simulink model "foc_simulink"  (R2022b)
settings: Solver=FixedStepDiscrete  StartTime=0.0  StopTime=0.5  RelTol=1e-3
InitFcn:
  | SPEED_PI_P=0.003
  | SPEED_PI_I=5
  | SPEED_PI_UP_LIMIT = 5.0
  | SPEED_PI_LOW_LIMIT = -5.0
  | SPEED_PI_KB = 0.015
  | D_PI_P = 1.4
  | D_PI_I = 600
  | D_PI_UP_LIMIT = 24.0
  | D_PI_LOW_LIMIT = -24.0
  | D_PI_KB = 15
  | Q_PI_P = 1.4
  | Q_PI_I = 600
  | Q_PI_UP_LIMIT = 24.0
  | Q_PI_LOW_LIMIT = -24.0
  | Q_PI_KB = 15
values from neighbouring files (symbols this model uses):
  L = 0.00046    [electric_current_loop.m]    (also in electric_kp_ki.m; pll.m = 10000; sl_ekf.m = c.L_LINE; sl_flux.m = L_avg - 0.5 * L_diff + L_diff * iq_obs * iq_obs / i2_obs)
libraries: slpidlib x8, spsPermanentMagnetSynchronousMachineLib x3, simulink x2, spsDCVoltageSourceLib x1, spsGroundLib x1, spsThreePhaseVIMeasurementLib x1, spsUniversalBridgeLib x1, sps_lib x1
(part 2 of 2)

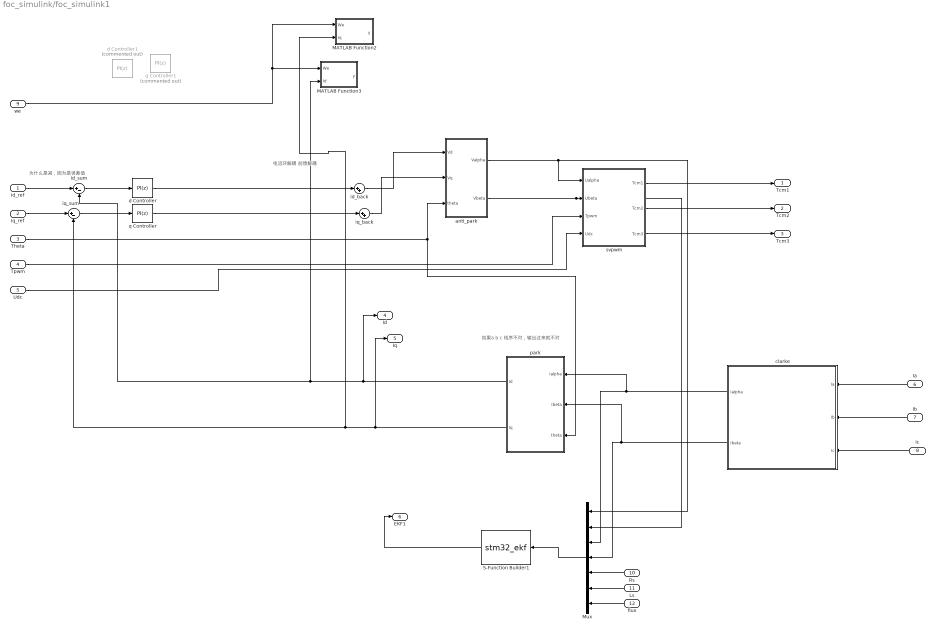
== system foc_simulink/foc_simulink1 ==
  note: 如果a b c 线序不对，输出过来就不对
  note: 为什么是减，因为是误差值
  note: 电流环解耦
      | 前馈解耦
  Id_ref : Inport
  Iq_ref : Inport  Port=2
  Theta : Inport  Port=3
  Tpwm : Inport  Port=4
  Udc : Inport  Port=5
  Ia : Inport  Port=6
  Ib : Inport  Port=7
  Ic : Inport  Port=8
  we : Inport  Port=9
  Rs : Inport  Port=10
  Ls : Inport  Port=11
  flux : Inport  Port=12
  MATLAB Function2 : MATLAB Function  TreatAsAtomicUnit=on
  MATLAB Function3 : MATLAB Function  TreatAsAtomicUnit=on
  Mux : Mux  Inputs=7
  S-Function Builder1 : S-Function  InitFcn=try, set_param(gcb,'FunctionName','stm32_ekf'), end  FunctionName=stm32_ekf  SFunctionModules=stm32_ekf_wrapper  SFunctionDeploymentMode=off  EnableBusSupport=off  mask(S-Function Builder){}
      mask help: Simulink:masks:SFunctionBuilder_MD
      mask init: same as foc_simulink/foc_simulink/EKF
      settings: CopyFcn=set_param(gcbh,'LinkStatus','none')  PreSaveFcn=try, set_param(gcb,'FunctionName','stm32_ekf'), end  OpenFcn=sfunctionwizard(gcbh)
      mask Display: plot(val(:,1),val(:,2)),disp(sys), port_label('input',1,'u'), port_label('output',1,'y')
  anti_park : Subsystem
  clarke : Subsystem
  d Controller : slpidlib/PID Controller  Controller=PI  Form=Parallel  TimeDomain=Discrete-time  UseExternalTs=off  SampleTime=-1  IntegratorMethod=Forward Euler  FilterMethod=Forward Euler  ControllerParametersSource=internal  P=D_PI_P  I=D_PI_I  UseKiTs=off  D=0.09  N=100  UseFilter=on  TunerSelectOption=Transfer Function Based (PID Tuner App)  InitialConditionSource=internal  InitialConditionForIntegrator=0  InitialConditionForFilter=0  DifferentiatorICPrevScaledInput=0  ExternalReset=none  TrackingMode=off  Kt=1  LimitOutput=on  SatLimitsSource=internal  UpperSaturationLimit=D_PI_UP_LIMIT  LowerSaturationLimit=D_PI_LOW_LIMIT  LinearizeAsGain=off  AntiWindupMode=back-calculation  Kb=D_PI_KB  LimitIntegrator=off  UpperIntegratorSaturationLimit=inf  LowerIntegratorSaturationLimit=-inf  PGainOutDataTypeStr=single  PProdOutDataTypeStr=single  POutMin=[]  POutMax=[]  IGainOutDataTypeStr=single  IProdOutDataTypeStr=single  IOutMin=[]  IOutMax=[]  DOutMin=[]  DOutMax=[]  NOutMin=[]  NOutMax=[]  SumOutDataTypeStr=single  SumOutMin=[]  SumOutMax=[]  SaturationOutDataTypeStr=single  SaturationOutMin=[]  SaturationOutMax=[]  PParamDataTypeStr=single  PParamMin=[]  PParamMax=[]  IParamDataTypeStr=single  IParamMin=[]  IParamMax=[]  DParamMin=[]  DParamMax=[]  NParamMin=[]  NParamMax=[]  KbParamDataTypeStr=single  KbParamMin=[]  KbParamMax=[]  KtParamMin=[]  KtParamMax=[]  KbOutDataTypeStr=single  KbOutMin=[]  KbOutMax=[]  KtOutMin=[]  KtOutMax=[]  IntegratorOutDataTypeStr=single  IntegratorOutMin=[]  IntegratorOutMax=[]  FilterOutMin=[]  FilterOutMax=[]  SumI1OutDataTypeStr=single  SumI1OutMin=[]  SumI1OutMax=[]  SumI2OutDataTypeStr=single  SumI2OutMin=[]  SumI2OutMax=[]  SumI3OutMin=[]  SumI3OutMax=[]  SumI4OutMin=[]  SumI4OutMax=[]  SumDOutMin=[]  SumDOutMax=[]  SumAccumDataTypeStr=single  SumI1AccumDataTypeStr=single  SumI2AccumDataTypeStr=single  DifferentiatorOutMin=[]  DifferentiatorOutMax=[]  FilterDiffOutCoefMin=[]  FilterDiffOutCoefMax=[]  ReciprocalOutMin=[]  ReciprocalOutMax=[]  SumDenOutMin=[]  SumDenOutMax=[]  SumNumOutMin=[]  SumNumOutMax=[]  DivideOutMin=[]  DivideOutMax=[]  UdiffTsProdOutMin=[]  UdiffTsProdOutMax=[]  NTsProdOutMin=[]  NTsProdOutMax=[]  UintegralTsProdOutMin=[]  UintegralTsProdOutMax=[]  UngainTsProdOutMin=[]  UngainTsProdOutMax=[]  ClampingZeroOutDataTypeStr=Inherit: Inherit via back propagation  ClampingZeroOutMin=[]  ClampingZeroOutMax=[]  FilterDenConstantOutDataTypeStr=Inherit: Inherit via back propagation  FilterDenConstantOutMin=[]  FilterDenConstantOutMax=[]  PCopyOutDataTypeStr=Inherit: Inherit via back propagation  PCopyOutMin=[]  PCopyOutMax=[]  NCopyOutDataTypeStr=Inherit: Inherit via back propagation  NCopyOutMin=[]  NCopyOutMax=[]  IntegratorContinuousStateAttributes=''  IntegratorStateIdentifier=di  IntegratorStateMustResolveToSignalObject=off  IntegratorRTWStateStorageClass=Auto  FilterContinuousStateAttributes=''  FilterStateMustResolveToSignalObject=off  FilterRTWStateStorageClass=Auto  ParallelPVariant=InternalParameters  IdealPVariant=Disabled  IVariant=InternalParameters  DVariant=Disabled  IntegratorVariant=Discrete  SatVariant=Enabled  AWVariant=BackCalculation  PCopyVariant=Disabled  TRVariant=Disabled  FdbkBlocksVariant=Forward  IdealPFdbkVariant=Disabled  SatFdbkVariant=Disabled  DerivativeFilterVariant=Disabled  NVariant=Disabled  NCopyVariant=Disabled_SignalSpec  FilterICVariant=Disabled  IntegratorICVariant=InternalICs  ExternalResetVariant=Disabled  TRSumVariant=Passthrough  SumFdbkVariant=Disabled  SumVariant=Sum_PI  TsampFilterVariant=InternalTs  TsampNgainVariant=Passthrough  TsampIntegralVariant=Passthrough  ExternalSaturationOutDataTypeStr=Inherit: Same as second input
  d Controller1 : slpidlib/PID Controller  Commented=on  Controller=PI  Form=Parallel  TimeDomain=Discrete-time  UseExternalTs=off  SampleTime=-1  IntegratorMethod=Forward Euler  FilterMethod=Forward Euler  ControllerParametersSource=internal  P=D_PI_P  I=D_PI_I  UseKiTs=off  D=0.09  N=100  UseFilter=on  TunerSelectOption=Transfer Function Based (PID Tuner App)  InitialConditionSource=internal  InitialConditionForIntegrator=0  InitialConditionForFilter=0  DifferentiatorICPrevScaledInput=0  ExternalReset=none  TrackingMode=off  Kt=1  LimitOutput=on  SatLimitsSource=internal  UpperSaturationLimit=D_PI_UP_LIMIT  LowerSaturationLimit=D_PI_LOW_LIMIT  LinearizeAsGain=off  AntiWindupMode=back-calculation  Kb=D_PI_KB  LimitIntegrator=off  UpperIntegratorSaturationLimit=inf  LowerIntegratorSaturationLimit=-inf  PGainOutDataTypeStr=single  PProdOutDataTypeStr=single  POutMin=[]  POutMax=[]  IGainOutDataTypeStr=single  IProdOutDataTypeStr=single  IOutMin=[]  IOutMax=[]  DOutMin=[]  DOutMax=[]  NOutMin=[]  NOutMax=[]  SumOutDataTypeStr=single  SumOutMin=[]  SumOutMax=[]  SaturationOutDataTypeStr=single  SaturationOutMin=[]  SaturationOutMax=[]  PParamDataTypeStr=single  PParamMin=[]  PParamMax=[]  IParamDataTypeStr=single  IParamMin=[]  IParamMax=[]  DParamMin=[]  DParamMax=[]  NParamMin=[]  NParamMax=[]  KbParamDataTypeStr=single  KbParamMin=[]  KbParamMax=[]  KtParamMin=[]  KtParamMax=[]  KbOutDataTypeStr=single  KbOutMin=[]  KbOutMax=[]  KtOutMin=[]  KtOutMax=[]  IntegratorOutDataTypeStr=single  IntegratorOutMin=[]  IntegratorOutMax=[]  FilterOutMin=[]  FilterOutMax=[]  SumI1OutDataTypeStr=single  SumI1OutMin=[]  SumI1OutMax=[]  SumI2OutDataTypeStr=single  SumI2OutMin=[]  SumI2OutMax=[]  SumI3OutMin=[]  SumI3OutMax=[]  SumI4OutMin=[]  SumI4OutMax=[]  SumDOutMin=[]  SumDOutMax=[]  SumAccumDataTypeStr=single  SumI1AccumDataTypeStr=single  SumI2AccumDataTypeStr=single  DifferentiatorOutMin=[]  DifferentiatorOutMax=[]  FilterDiffOutCoefMin=[]  FilterDiffOutCoefMax=[]  ReciprocalOutMin=[]  ReciprocalOutMax=[]  SumDenOutMin=[]  SumDenOutMax=[]  SumNumOutMin=[]  SumNumOutMax=[]  DivideOutMin=[]  DivideOutMax=[]  UdiffTsProdOutMin=[]  UdiffTsProdOutMax=[]  NTsProdOutMin=[]  NTsProdOutMax=[]  UintegralTsProdOutMin=[]  UintegralTsProdOutMax=[]  UngainTsProdOutMin=[]  UngainTsProdOutMax=[]  ClampingZeroOutDataTypeStr=Inherit: Inherit via back propagation  ClampingZeroOutMin=[]  ClampingZeroOutMax=[]  FilterDenConstantOutDataTypeStr=Inherit: Inherit via back propagation  FilterDenConstantOutMin=[]  FilterDenConstantOutMax=[]  PCopyOutDataTypeStr=Inherit: Inherit via back propagation  PCopyOutMin=[]  PCopyOutMax=[]  NCopyOutDataTypeStr=Inherit: Inherit via back propagation  NCopyOutMin=[]  NCopyOutMax=[]  IntegratorContinuousStateAttributes=''  IntegratorStateIdentifier=di  IntegratorStateMustResolveToSignalObject=off  IntegratorRTWStateStorageClass=Auto  FilterContinuousStateAttributes=''  FilterStateMustResolveToSignalObject=off  FilterRTWStateStorageClass=Auto  ParallelPVariant=InternalParameters  IdealPVariant=Disabled  IVariant=InternalParameters  DVariant=Disabled  IntegratorVariant=Discrete  SatVariant=Enabled  AWVariant=BackCalculation  PCopyVariant=Disabled  TRVariant=Disabled  FdbkBlocksVariant=Forward  IdealPFdbkVariant=Disabled  SatFdbkVariant=Disabled  DerivativeFilterVariant=Disabled  NVariant=Disabled  NCopyVariant=Disabled_SignalSpec  FilterICVariant=Disabled  IntegratorICVariant=InternalICs  ExternalResetVariant=Disabled  TRSumVariant=Passthrough  SumFdbkVariant=Disabled  SumVariant=Sum_PI  TsampFilterVariant=InternalTs  TsampNgainVariant=Passthrough  TsampIntegralVariant=Passthrough  ExternalSaturationOutDataTypeStr=Inherit: Same as second input
  id_back : Sum  Inputs=|++
  id_sum : Sum  Inputs=|+-
  iq_back : Sum  Inputs=|++
  iq_sum : Sum  Inputs=|+-
  park : Subsystem
  q Controller : slpidlib/PID Controller  Controller=PI  Form=Parallel  TimeDomain=Discrete-time  UseExternalTs=off  SampleTime=-1  IntegratorMethod=Forward Euler  FilterMethod=Forward Euler  ControllerParametersSource=internal  P=Q_PI_P  I=Q_PI_I  UseKiTs=off  D=0.09  N=100  UseFilter=on  TunerSelectOption=Transfer Function Based (PID Tuner App)  InitialConditionSource=internal  InitialConditionForIntegrator=0  InitialConditionForFilter=0  DifferentiatorICPrevScaledInput=0  ExternalReset=none  TrackingMode=off  Kt=1  LimitOutput=on  SatLimitsSource=internal  UpperSaturationLimit=Q_PI_UP_LIMIT  LowerSaturationLimit=Q_PI_LOW_LIMIT  LinearizeAsGain=off  AntiWindupMode=back-calculation  Kb=Q_PI_KB  LimitIntegrator=off  UpperIntegratorSaturationLimit=inf  LowerIntegratorSaturationLimit=-inf  PGainOutDataTypeStr=single  PProdOutDataTypeStr=single  POutMin=[]  POutMax=[]  IGainOutDataTypeStr=single  IProdOutDataTypeStr=single  IOutMin=[]  IOutMax=[]  DOutMin=[]  DOutMax=[]  NOutMin=[]  NOutMax=[]  SumOutDataTypeStr=single  SumOutMin=[]  SumOutMax=[]  SaturationOutDataTypeStr=single  SaturationOutMin=[]  SaturationOutMax=[]  PParamDataTypeStr=single  PParamMin=[]  PParamMax=[]  IParamDataTypeStr=single  IParamMin=[]  IParamMax=[]  DParamMin=[]  DParamMax=[]  NParamMin=[]  NParamMax=[]  KbParamDataTypeStr=single  KbParamMin=[]  KbParamMax=[]  KtParamMin=[]  KtParamMax=[]  KbOutDataTypeStr=single  KbOutMin=[]  KbOutMax=[]  KtOutMin=[]  KtOutMax=[]  IntegratorOutDataTypeStr=single  IntegratorOutMin=[]  IntegratorOutMax=[]  FilterOutMin=[]  FilterOutMax=[]  SumI1OutDataTypeStr=single  SumI1OutMin=[]  SumI1OutMax=[]  SumI2OutDataTypeStr=single  SumI2OutMin=[]  SumI2OutMax=[]  SumI3OutMin=[]  SumI3OutMax=[]  SumI4OutMin=[]  SumI4OutMax=[]  SumDOutMin=[]  SumDOutMax=[]  SumAccumDataTypeStr=single  SumI1AccumDataTypeStr=single  SumI2AccumDataTypeStr=single  DifferentiatorOutMin=[]  DifferentiatorOutMax=[]  FilterDiffOutCoefMin=[]  FilterDiffOutCoefMax=[]  ReciprocalOutMin=[]  ReciprocalOutMax=[]  SumDenOutMin=[]  SumDenOutMax=[]  SumNumOutMin=[]  SumNumOutMax=[]  DivideOutMin=[]  DivideOutMax=[]  UdiffTsProdOutMin=[]  UdiffTsProdOutMax=[]  NTsProdOutMin=[]  NTsProdOutMax=[]  UintegralTsProdOutMin=[]  UintegralTsProdOutMax=[]  UngainTsProdOutMin=[]  UngainTsProdOutMax=[]  ClampingZeroOutDataTypeStr=Inherit: Inherit via back propagation  ClampingZeroOutMin=[]  ClampingZeroOutMax=[]  FilterDenConstantOutDataTypeStr=Inherit: Inherit via back propagation  FilterDenConstantOutMin=[]  FilterDenConstantOutMax=[]  PCopyOutDataTypeStr=Inherit: Inherit via back propagation  PCopyOutMin=[]  PCopyOutMax=[]  NCopyOutDataTypeStr=Inherit: Inherit via back propagation  NCopyOutMin=[]  NCopyOutMax=[]  IntegratorContinuousStateAttributes=''  IntegratorStateIdentifier=qi  IntegratorStateMustResolveToSignalObject=off  IntegratorRTWStateStorageClass=Auto  FilterContinuousStateAttributes=''  FilterStateMustResolveToSignalObject=off  FilterRTWStateStorageClass=Auto  ParallelPVariant=InternalParameters  IdealPVariant=Disabled  IVariant=InternalParameters  DVariant=Disabled  IntegratorVariant=Discrete  SatVariant=Enabled  AWVariant=BackCalculation  PCopyVariant=Disabled  TRVariant=Disabled  FdbkBlocksVariant=Forward  IdealPFdbkVariant=Disabled  SatFdbkVariant=Disabled  DerivativeFilterVariant=Disabled  NVariant=Disabled  NCopyVariant=Disabled_SignalSpec  FilterICVariant=Disabled  IntegratorICVariant=InternalICs  ExternalResetVariant=Disabled  TRSumVariant=Passthrough  SumFdbkVariant=Disabled  SumVariant=Sum_PI  TsampFilterVariant=InternalTs  TsampNgainVariant=Passthrough  TsampIntegralVariant=Passthrough  ExternalSaturationOutDataTypeStr=Inherit: Same as second input
  q Controller1 : slpidlib/PID Controller  Commented=on  Controller=PI  Form=Parallel  TimeDomain=Discrete-time  UseExternalTs=off  SampleTime=-1  IntegratorMethod=Forward Euler  FilterMethod=Forward Euler  ControllerParametersSource=internal  P=Q_PI_P  I=Q_PI_I  UseKiTs=off  D=0.09  N=100  UseFilter=on  TunerSelectOption=Transfer Function Based (PID Tuner App)  InitialConditionSource=internal  InitialConditionForIntegrator=0  InitialConditionForFilter=0  DifferentiatorICPrevScaledInput=0  ExternalReset=none  TrackingMode=off  Kt=1  LimitOutput=on  SatLimitsSource=internal  UpperSaturationLimit=Q_PI_UP_LIMIT  LowerSaturationLimit=Q_PI_LOW_LIMIT  LinearizeAsGain=off  AntiWindupMode=back-calculation  Kb=Q_PI_KB  LimitIntegrator=off  UpperIntegratorSaturationLimit=inf  LowerIntegratorSaturationLimit=-inf  PGainOutDataTypeStr=single  PProdOutDataTypeStr=single  POutMin=[]  POutMax=[]  IGainOutDataTypeStr=single  IProdOutDataTypeStr=single  IOutMin=[]  IOutMax=[]  DOutMin=[]  DOutMax=[]  NOutMin=[]  NOutMax=[]  SumOutDataTypeStr=single  SumOutMin=[]  SumOutMax=[]  SaturationOutDataTypeStr=single  SaturationOutMin=[]  SaturationOutMax=[]  PParamDataTypeStr=single  PParamMin=[]  PParamMax=[]  IParamDataTypeStr=single  IParamMin=[]  IParamMax=[]  DParamMin=[]  DParamMax=[]  NParamMin=[]  NParamMax=[]  KbParamDataTypeStr=single  KbParamMin=[]  KbParamMax=[]  KtParamMin=[]  KtParamMax=[]  KbOutDataTypeStr=single  KbOutMin=[]  KbOutMax=[]  KtOutMin=[]  KtOutMax=[]  IntegratorOutDataTypeStr=single  IntegratorOutMin=[]  IntegratorOutMax=[]  FilterOutMin=[]  FilterOutMax=[]  SumI1OutDataTypeStr=single  SumI1OutMin=[]  SumI1OutMax=[]  SumI2OutDataTypeStr=single  SumI2OutMin=[]  SumI2OutMax=[]  SumI3OutMin=[]  SumI3OutMax=[]  SumI4OutMin=[]  SumI4OutMax=[]  SumDOutMin=[]  SumDOutMax=[]  SumAccumDataTypeStr=single  SumI1AccumDataTypeStr=single  SumI2AccumDataTypeStr=single  DifferentiatorOutMin=[]  DifferentiatorOutMax=[]  FilterDiffOutCoefMin=[]  FilterDiffOutCoefMax=[]  ReciprocalOutMin=[]  ReciprocalOutMax=[]  SumDenOutMin=[]  SumDenOutMax=[]  SumNumOutMin=[]  SumNumOutMax=[]  DivideOutMin=[]  DivideOutMax=[]  UdiffTsProdOutMin=[]  UdiffTsProdOutMax=[]  NTsProdOutMin=[]  NTsProdOutMax=[]  UintegralTsProdOutMin=[]  UintegralTsProdOutMax=[]  UngainTsProdOutMin=[]  UngainTsProdOutMax=[]  ClampingZeroOutDataTypeStr=Inherit: Inherit via back propagation  ClampingZeroOutMin=[]  ClampingZeroOutMax=[]  FilterDenConstantOutDataTypeStr=Inherit: Inherit via back propagation  FilterDenConstantOutMin=[]  FilterDenConstantOutMax=[]  PCopyOutDataTypeStr=Inherit: Inherit via back propagation  PCopyOutMin=[]  PCopyOutMax=[]  NCopyOutDataTypeStr=Inherit: Inherit via back propagation  NCopyOutMin=[]  NCopyOutMax=[]  IntegratorContinuousStateAttributes=''  IntegratorStateIdentifier=qi  IntegratorStateMustResolveToSignalObject=off  IntegratorRTWStateStorageClass=Auto  FilterContinuousStateAttributes=''  FilterStateMustResolveToSignalObject=off  FilterRTWStateStorageClass=Auto  ParallelPVariant=InternalParameters  IdealPVariant=Disabled  IVariant=InternalParameters  DVariant=Disabled  IntegratorVariant=Discrete  SatVariant=Enabled  AWVariant=BackCalculation  PCopyVariant=Disabled  TRVariant=Disabled  FdbkBlocksVariant=Forward  IdealPFdbkVariant=Disabled  SatFdbkVariant=Disabled  DerivativeFilterVariant=Disabled  NVariant=Disabled  NCopyVariant=Disabled_SignalSpec  FilterICVariant=Disabled  IntegratorICVariant=InternalICs  ExternalResetVariant=Disabled  TRSumVariant=Passthrough  SumFdbkVariant=Disabled  SumVariant=Sum_PI  TsampFilterVariant=InternalTs  TsampNgainVariant=Passthrough  TsampIntegralVariant=Passthrough  ExternalSaturationOutDataTypeStr=Inherit: Same as second input
  svpwm : Subsystem
  Tcm1 : Outport
  Tcm2 : Outport  Port=2
  Tcm3 : Outport  Port=3
  Id : Outport  Port=4
  Iq : Outport  Port=5
  EKF1 : Outport  Port=6  VectorParamsAs1DForOutWhenUnconnected=off
  wires:
  flux/1 -> Mux/7
  S-Function Builder1/1 -> EKF1/1
  anti_park/2(Vbeta) -> svpwm/2(Ubeta), Mux/2
  clarke/2(Ibeta) -> park/2(Ibeta), Mux/4
  clarke/1(Ialpha) -> Mux/3, park/1(Ialpha)
  Mux/1 -> S-Function Builder1/1
  anti_park/1(Valpha) -> svpwm/1(Ualpha), Mux/1
  Rs/1 -> Mux/5
  Ls/1 -> Mux/6
  iq_back/1 -> anti_park/2(Vq)
  id_back/1 -> anti_park/1(Vd)
  d Controller/1 -> id_back/1
  id_sum/1 -> d Controller/1
  Id_ref/1 -> id_sum/1
  q Controller/1 -> iq_back/1
  we/1 -> MATLAB Function2/1(We), MATLAB Function3/1(We)
  iq_sum/1 -> q Controller/1
  Iq_ref/1 -> iq_sum/1
  park/2(Iq) -> iq_sum/2, MATLAB Function2/2(Iq), Iq/1
  park/1(Id) -> id_sum/2, MATLAB Function3/2(Id), Id/1
  Ic/1 -> clarke/3(Ic)
  Ib/1 -> clarke/2(Ib)
  Ia/1 -> clarke/1(Ia)
  svpwm/2(Tcm2) -> Tcm2/1
  svpwm/1(Tcm1) -> Tcm1/1
  svpwm/3(Tcm3) -> Tcm3/1
  Tpwm/1 -> svpwm/3(Tpwm)
  Udc/1 -> svpwm/4(Udc)
  Theta/1 -> park/3(theta), anti_park/3(theta)

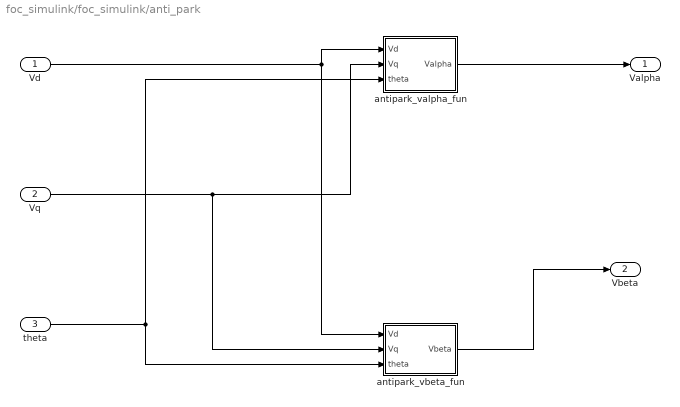
== system foc_simulink/foc_simulink/anti_park ==
  Vd : Inport
  Vq : Inport  Port=2
  theta : Inport  Port=3
  antipark_valpha_fun : MATLAB Function  TreatAsAtomicUnit=on
  antipark_vbeta_fun : MATLAB Function  TreatAsAtomicUnit=on
  Valpha : Outport
  Vbeta : Outport  Port=2
  wires:
  antipark_valpha_fun/1(Valpha) -> Valpha/1
  antipark_vbeta_fun/1(Vbeta) -> Vbeta/1
  Vd/1 -> antipark_valpha_fun/1(Vd), antipark_vbeta_fun/1(Vd)
  Vq/1 -> antipark_valpha_fun/2(Vq), antipark_vbeta_fun/2(Vq)
  theta/1 -> antipark_valpha_fun/3(theta), antipark_vbeta_fun/3(theta)

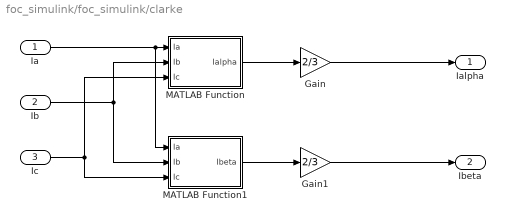
== system foc_simulink/foc_simulink/clarke ==
  Ia : Inport
  Ib : Inport  Port=2
  Ic : Inport  Port=3
  Gain : Gain  Gain=2/3  OutDataTypeStr=single
  Gain1 : Gain  Gain=2/3  OutDataTypeStr=single
  MATLAB Function : MATLAB Function  TreatAsAtomicUnit=on
  MATLAB Function1 : MATLAB Function  TreatAsAtomicUnit=on
  Ialpha : Outport
  Ibeta : Outport  Port=2
  wires:
  Ia/1 -> MATLAB Function1/1(Ia), MATLAB Function/1(Ia)
  MATLAB Function/1(Ialpha) -> Gain/1
  Gain1/1 -> Ibeta/1
  Ib/1 -> MATLAB Function1/2(Ib), MATLAB Function/2(Ib)
  Ic/1 -> MATLAB Function/3(Ic), MATLAB Function1/3(Ic)
  MATLAB Function1/1(Ibeta) -> Gain1/1
  Gain/1 -> Ialpha/1

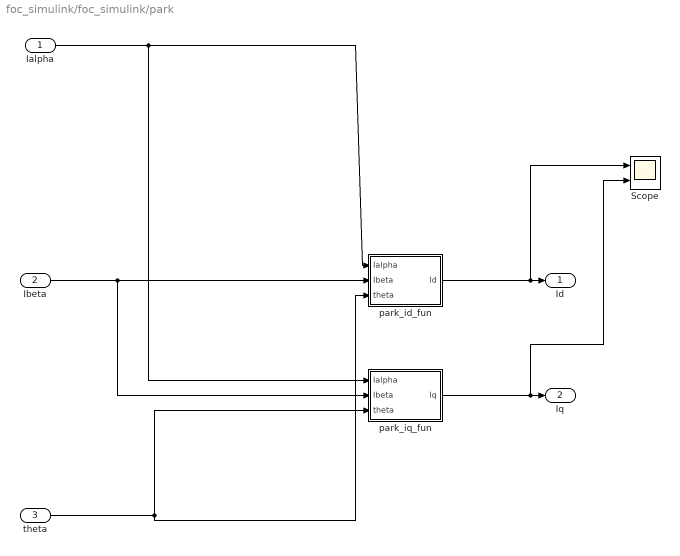
== system foc_simulink/foc_simulink/park ==
  Ialpha : Inport
  Ibeta : Inport  Port=2
  theta : Inport  Port=3
  Scope : Scope  NumInputPorts=2
  park_id_fun : MATLAB Function  TreatAsAtomicUnit=on
  park_iq_fun : MATLAB Function  TreatAsAtomicUnit=on
  Id : Outport
  Iq : Outport  Port=2
  wires:
  theta/1 -> park_id_fun/3(theta), park_iq_fun/3(theta)
  Ibeta/1 -> park_id_fun/2(Ibeta), park_iq_fun/2(Ibeta)
  park_iq_fun/1(Iq) -> Scope/2, Iq/1
  park_id_fun/1(Id) -> Scope/1, Id/1
  Ialpha/1 -> park_id_fun/1(Ialpha), park_iq_fun/1(Ialpha)

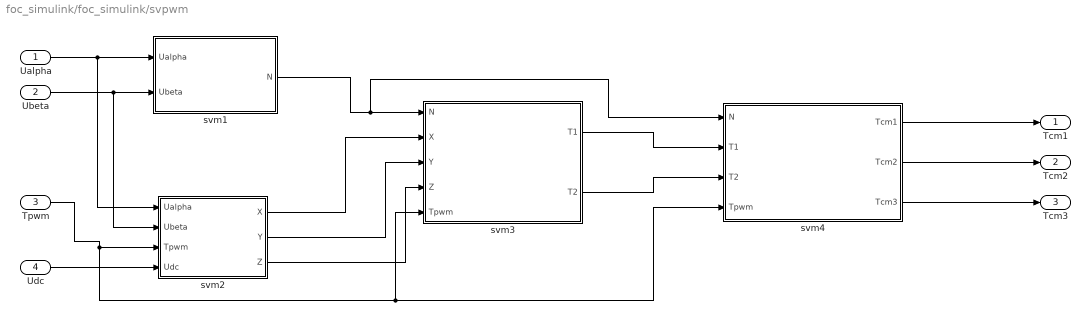
== system foc_simulink/foc_simulink/svpwm ==
  Ualpha : Inport
  Ubeta : Inport  Port=2
  Tpwm : Inport  Port=3
  Udc : Inport  Port=4
  svm1 : MATLAB Function  TreatAsAtomicUnit=on
  svm2 : MATLAB Function  TreatAsAtomicUnit=on
  svm3 : MATLAB Function  TreatAsAtomicUnit=on
  svm4 : MATLAB Function  TreatAsAtomicUnit=on
  Tcm1 : Outport
  Tcm2 : Outport  Port=2
  Tcm3 : Outport  Port=3
  wires:
  svm4/2(Tcm2) -> Tcm2/1
  Tpwm/1 -> svm4/4(Tpwm), svm3/5(Tpwm), svm2/3(Tpwm)
  svm1/1(N) -> svm4/1(N), svm3/1(N)
  Udc/1 -> svm2/4(Udc)
  svm4/3(Tcm3) -> Tcm3/1
  svm3/1(T1) -> svm4/2(T1)
  Ualpha/1 -> svm2/1(Ualpha), svm1/1(Ualpha)
  svm3/2(T2) -> svm4/3(T2)
  Ubeta/1 -> svm2/2(Ubeta), svm1/2(Ubeta)
  svm4/1(Tcm1) -> Tcm1/1
  svm2/1(X) -> svm3/2(X)
  svm2/3(Z) -> svm3/4(Z)
  svm2/2(Y) -> svm3/3(Y)

== system foc_simulink/foc_simulink1/anti_park ==
  Vd : Inport
  Vq : Inport  Port=2
  theta : Inport  Port=3
  antipark_valpha_fun : MATLAB Function  TreatAsAtomicUnit=on
  antipark_vbeta_fun : MATLAB Function  TreatAsAtomicUnit=on
  Valpha : Outport
  Vbeta : Outport  Port=2
  wires:
  theta/1 -> antipark_vbeta_fun/3(theta), antipark_valpha_fun/3(theta)
  Vq/1 -> antipark_vbeta_fun/2(Vq), antipark_valpha_fun/2(Vq)
  Vd/1 -> antipark_vbeta_fun/1(Vd), antipark_valpha_fun/1(Vd)
  antipark_vbeta_fun/1(Vbeta) -> Vbeta/1
  antipark_valpha_fun/1(Valpha) -> Valpha/1

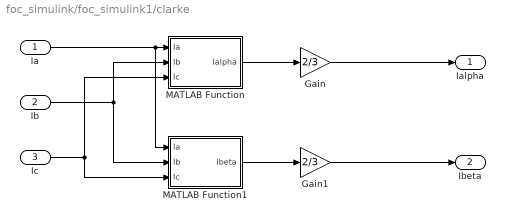
== system foc_simulink/foc_simulink1/clarke ==
  Ia : Inport
  Ib : Inport  Port=2
  Ic : Inport  Port=3
  Gain : Gain  Gain=2/3  OutDataTypeStr=single
  Gain1 : Gain  Gain=2/3  OutDataTypeStr=single
  MATLAB Function : MATLAB Function  TreatAsAtomicUnit=on
  MATLAB Function1 : MATLAB Function  TreatAsAtomicUnit=on
  Ialpha : Outport
  Ibeta : Outport  Port=2
  wires:
  Gain/1 -> Ialpha/1
  MATLAB Function1/1(Ibeta) -> Gain1/1
  Ic/1 -> MATLAB Function1/3(Ic), MATLAB Function/3(Ic)
  Ib/1 -> MATLAB Function/2(Ib), MATLAB Function1/2(Ib)
  Gain1/1 -> Ibeta/1
  MATLAB Function/1(Ialpha) -> Gain/1
  Ia/1 -> MATLAB Function/1(Ia), MATLAB Function1/1(Ia)

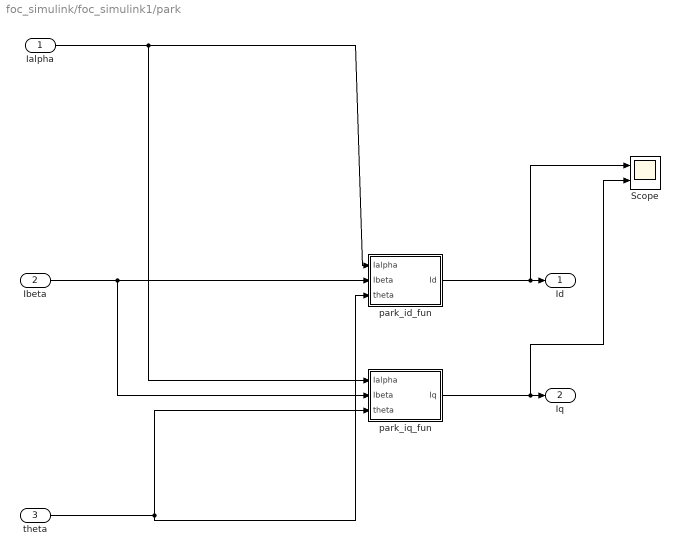
== system foc_simulink/foc_simulink1/park ==
  Ialpha : Inport
  Ibeta : Inport  Port=2
  theta : Inport  Port=3
  Scope : Scope  NumInputPorts=2
  park_id_fun : MATLAB Function  TreatAsAtomicUnit=on
  park_iq_fun : MATLAB Function  TreatAsAtomicUnit=on
  Id : Outport
  Iq : Outport  Port=2
  wires:
  Ialpha/1 -> park_iq_fun/1(Ialpha), park_id_fun/1(Ialpha)
  park_id_fun/1(Id) -> Id/1, Scope/1
  park_iq_fun/1(Iq) -> Iq/1, Scope/2
  Ibeta/1 -> park_iq_fun/2(Ibeta), park_id_fun/2(Ibeta)
  theta/1 -> park_iq_fun/3(theta), park_id_fun/3(theta)

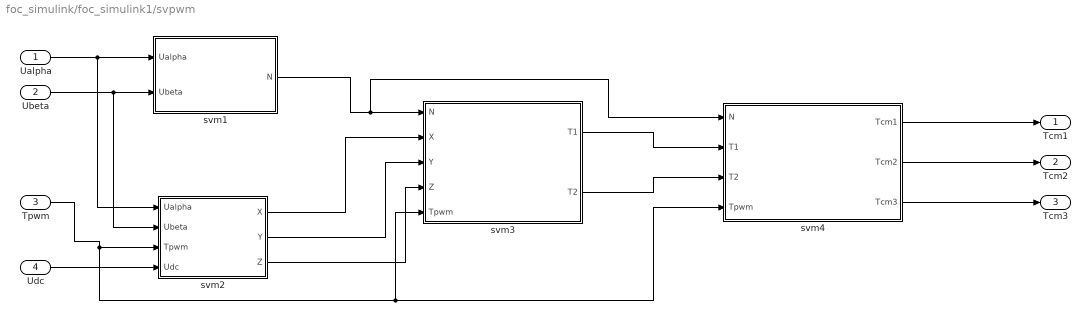
== system foc_simulink/foc_simulink1/svpwm ==
  Ualpha : Inport
  Ubeta : Inport  Port=2
  Tpwm : Inport  Port=3
  Udc : Inport  Port=4
  svm1 : MATLAB Function  TreatAsAtomicUnit=on
  svm2 : MATLAB Function  TreatAsAtomicUnit=on
  svm3 : MATLAB Function  TreatAsAtomicUnit=on
  svm4 : MATLAB Function  TreatAsAtomicUnit=on
  Tcm1 : Outport
  Tcm2 : Outport  Port=2
  Tcm3 : Outport  Port=3
  wires:
  svm2/2(Y) -> svm3/3(Y)
  svm2/3(Z) -> svm3/4(Z)
  svm2/1(X) -> svm3/2(X)
  svm4/1(Tcm1) -> Tcm1/1
  Ubeta/1 -> svm1/2(Ubeta), svm2/2(Ubeta)
  svm3/2(T2) -> svm4/3(T2)
  Ualpha/1 -> svm1/1(Ualpha), svm2/1(Ualpha)
  svm3/1(T1) -> svm4/2(T1)
  svm4/3(Tcm3) -> Tcm3/1
  Udc/1 -> svm2/4(Udc)
  svm1/1(N) -> svm3/1(N), svm4/1(N)
  Tpwm/1 -> svm2/3(Tpwm), svm3/5(Tpwm), svm4/4(Tpwm)
  svm4/2(Tcm2) -> Tcm2/1

== matlab function foc_simulink/svpwm/svm4 ==
  data: N input; Tcm1 output; T1 input; T2 input; Tpwm input; Tcm2 output; Tcm3 output
function [Tcm1, Tcm2, Tcm3] = fcn(N, T1, T2, Tpwm)

Tcm1 = single(0);
Tcm2 = single(0);
Tcm3 = single(0);


if N == 1
    Tcm1 = (Tpwm + T1 - T2) / 4;
    Tcm2 = (Tpwm - T1 - T2) / 4;
    Tcm3 = (Tpwm + T1 + T2) / 4;
elseif N == 2
    Tcm1 = (Tpwm - T1 - T2) / 4;
    Tcm2 = (Tpwm + T1 + T2) / 4;
    Tcm3 = (Tpwm + T1 - T2) / 4;
elseif N == 3
    Tcm1 = (Tpwm - T1 - T2) / 4;
    Tcm2 = (Tpwm + T1 - T2) / 4;
    Tcm3 = (Tpwm + T1 + T2) / 4;
elseif N == 4
    Tcm1 = (Tpwm + T1 + T2) / 4;
    Tcm2 = (Tpwm + T1 - T2) / 4;
    Tcm3 = (Tpwm - T1 - T2) / 4;
elseif N == 5
    Tcm1 = (Tpwm + T1 + T2) / 4;
    Tcm2 = (Tpwm - T1 - T2) / 4;
    Tcm3 = (Tpwm + T1 - T2) / 4;
elseif N == 6
    Tcm1 = (Tpwm + T1 - T2) / 4;
    Tcm2 = (Tpwm + T1 + T2) / 4;
    Tcm3 = (Tpwm - T1 - T2) / 4;
end

== matlab function foc_simulink/clarke/MATLAB Function1 ==
  data: Ia input; Ibeta output; Ib input; Ic input
function Ibeta = fcn( Ia, Ib, Ic)

Ibeta = sqrt(3)/2 * (Ia + 2 * Ib);

== matlab function foc_simulink/MATLAB Function2 ==
  data: We input; y output; Iq input
function y = fcn(We, Iq)

% y = -We * Lq * Iq;
y = -We * 1.4e-3 * Iq;

== matlab function foc_simulink/MATLAB Function3 ==
  data: We input; y output; Id input
function y = fcn(We, Id)

% y = We * (Flux + Ld * Id);  
y = We * (0.034182 + 1.4e-3 * Id);

== matlab function foc_simulink/anti_park/antipark_vbeta_fun ==
  data: Vd input; Vbeta output; Vq input; theta input
function Vbeta = fcn(Vd, Vq, theta)

Vbeta = Vd * sin(theta) + Vq * cos(theta);

== matlab function foc_simulink/foc_simulink1/anti_park/antipark_valpha_fun ==
  data: Vd input; Valpha output; Vq input; theta input
function Valpha = fcn(Vd, Vq, theta)

Valpha = Vd * cos(theta) - Vq * sin(theta);

== matlab function foc_simulink/foc_simulink1/anti_park/antipark_vbeta_fun ==
  data: Vd input; Vbeta output; Vq input; theta input
function Vbeta = fcn(Vd, Vq, theta)

Vbeta = Vd * sin(theta) + Vq * cos(theta);

== matlab function foc_simulink/foc_simulink1/clarke/MATLAB Function ==
  data: Ia input; Ialpha output; Ib input; Ic input
function Ialpha = fcn(Ia, Ib, Ic)

Ialpha = 3/2 * Ia;

== matlab function foc_simulink/foc_simulink1/clarke/MATLAB Function1 ==
  data: Ia input; Ibeta output; Ib input; Ic input
function Ibeta = fcn( Ia, Ib, Ic)

Ibeta = sqrt(3)/2 * (Ia + 2 * Ib);

== matlab function foc_simulink/foc_simulink1/park/park_id_fun ==
  data: Ialpha input; Id output; Ibeta input; theta input
function Id = fcn(Ialpha, Ibeta, theta)

Id = Ialpha * cos(theta) + Ibeta * sin(theta);

== matlab function foc_simulink/foc_simulink1/park/park_iq_fun ==
  data: Ialpha input; Iq output; Ibeta input; theta input
function Iq = fcn(Ialpha, Ibeta, theta)
Iq = -Ialpha * sin(theta) + Ibeta * cos(theta);

== matlab function foc_simulink/foc_simulink1/svpwm/svm1 ==
  data: Ualpha input; N output; Ubeta input
function N = fcn(Ualpha, Ubeta)

U1 = Ubeta;
U2 = sqrt(3) * Ualpha - Ubeta;
U3 = -sqrt(3) * Ualpha - Ubeta;
A = 0;
B = 0;
C = 0;

if U1 > 0
    A = 1;
else
    A = 0;
end

if U2 > 0
    B = 1;
else
    B = 0;
end

if U3 > 0
    C = 1;
else
    C = 0;
end

N = A + 2 * B + 4 * C;

== matlab function foc_simulink/foc_simulink1/svpwm/svm2 ==
  data: Ualpha input; Ubeta input; Tpwm input; Udc input; X output; Y output; Z output
function [X, Y, Z] = fcn(Ualpha, Ubeta, Tpwm, Udc)

X = sqrt(3) * Tpwm * Ubeta / Udc;
Y = sqrt(3) * Tpwm / Udc * (sqrt(3) / 2 * Ualpha + 1 / 2 * Ubeta);
Z = sqrt(3) * Tpwm / Udc * (-sqrt(3) / 2 * Ualpha + 1 / 2 * Ubeta);

== matlab function foc_simulink/park/park_id_fun ==
  data: Ialpha input; Id output; Ibeta input; theta input
function Id = fcn(Ialpha, Ibeta, theta)

Id = -(Ialpha * cos(theta) + Ibeta * sin(theta));

== matlab function foc_simulink/anti_park/antipark_valpha_fun ==
  data: Vd input; Valpha output; Vq input; theta input
function Valpha = fcn(Vd, Vq, theta)

Valpha = Vd * cos(theta) - Vq * sin(theta);

== matlab function foc_simulink/park/park_iq_fun ==
  data: Ialpha input; Iq output; Ibeta input; theta input
function Iq = fcn(Ialpha, Ibeta, theta)
Iq = -(-Ialpha * sin(theta) + Ibeta * cos(theta));

== matlab function foc_simulink/foc_simulink1/svpwm/svm3 ==
  data: N input; T1 output; X input; Y input; Z input; Tpwm input; T2 output
function [T1, T2] = fcn(N, X, Y, Z, Tpwm)

T1 = single(0);
T2 = single(0);

if N == 1
    T1 = Z;
    T2 = Y;
elseif N == 2
    T1 = Y;
    T2 = -X;
elseif N == 3
    T1 = -Z;
    T2 = X;
elseif N == 4
    T1 = -X;
    T2 = Z;
elseif N == 5
    T1 = X;
    T2 = -Y;
elseif N == 6
    T1 = -Y;
    T2 = -Z;
end

== matlab function foc_simulink/foc_simulink1/svpwm/svm4 ==
  data: N input; Tcm1 output; T1 input; T2 input; Tpwm input; Tcm2 output; Tcm3 output
function [Tcm1, Tcm2, Tcm3] = fcn(N, T1, T2, Tpwm)

Tcm1 = single(0);
Tcm2 = single(0);
Tcm3 = single(0);


if N == 1
    Tcm1 = (Tpwm + T1 - T2) / 4;
    Tcm2 = (Tpwm - T1 - T2) / 4;
    Tcm3 = (Tpwm + T1 + T2) / 4;
elseif N == 2
    Tcm1 = (Tpwm - T1 - T2) / 4;
    Tcm2 = (Tpwm + T1 + T2) / 4;
    Tcm3 = (Tpwm + T1 - T2) / 4;
elseif N == 3
    Tcm1 = (Tpwm - T1 - T2) / 4;
    Tcm2 = (Tpwm + T1 - T2) / 4;
    Tcm3 = (Tpwm + T1 + T2) / 4;
elseif N == 4
    Tcm1 = (Tpwm + T1 + T2) / 4;
    Tcm2 = (Tpwm + T1 - T2) / 4;
    Tcm3 = (Tpwm - T1 - T2) / 4;
elseif N == 5
    Tcm1 = (Tpwm + T1 + T2) / 4;
    Tcm2 = (Tpwm - T1 - T2) / 4;
    Tcm3 = (Tpwm + T1 - T2) / 4;
elseif N == 6
    Tcm1 = (Tpwm + T1 - T2) / 4;
    Tcm2 = (Tpwm + T1 + T2) / 4;
    Tcm3 = (Tpwm - T1 - T2) / 4;
end

== matlab function foc_simulink/Subsystem1/SVPWM ==
  data: Alpha input; A output; B output; C output; Sector output; Beta input; PWMFullDutyCycle input
function [A, B, C, Sector] = fcn(Alpha, Beta, PWMFullDutyCycle)

% 初始化变量
A = single(0);
B = single(0);
C = single(0);                                  
Sector = 0;
ONE_BY_SQRT3 = tand(30);
TWO_BY_SQRT3 = (2.0 * 0.57735026919);

% 扇区判断
if Beta >= 0.0
    if Alpha >= 0.0
        if (ONE_BY_SQRT3 * Beta) > Alpha
                Sector = 2;
        else
            Sector = 1;
        end
    else
        if -ONE_BY_SQRT3 * Beta > Alpha
            Sector = 3;
        else
            Sector = 2;
        end
    end
else
    if Alpha >= 0.0
        if -ONE_BY_SQRT3 * Beta > Alpha
            Sector = 5;
        else
            Sector = 6;
        end

    else
        if ONE_BY_SQRT3 * Beta > Alpha
            Sector = 4;
        else
            Sector = 5;
        end
    end
end


switch Sector
    case 1
        t1 = (Alpha - ONE_BY_SQRT3 * Beta) * PWMFullDutyCycle;
        t2 = (TWO_BY_SQRT3 * Beta) * PWMFullDutyCycle;

        A = (PWMFullDutyCycle + t1 + t2) / 2;
        B = A - t1;
        C = B - t2;
    case 2
		t2 = (Alpha + ONE_BY_SQRT3 * Beta) * PWMFullDutyCycle;
		t3 = (-Alpha + ONE_BY_SQRT3 * Beta) * PWMFullDutyCycle;

		B = (PWMFullDutyCycle + t2 + t3) / 2;
		A = B - t3;
		C = A - t2;
        
    case 3
       t3 = (TWO_BY_SQRT3 * Beta) * PWMFullDutyCycle;
		t4 = (-Alpha - ONE_BY_SQRT3 * Beta) * PWMFullDutyCycle;

		B = (PWMFullDutyCycle + t3 + t4) / 2;
		C = B - t3;
		A = C - t4;

    case 4
		t4 = (-Alpha + ONE_BY_SQRT3 * Beta) * PWMFullDutyCycle;
		t5 = (-TWO_BY_SQRT3 * Beta) * PWMFullDutyCycle;

		C = (PWMFullDutyCycle + t4 + t5) / 2;
		B = C - t5;
		A = B - t4;
    case 5
        t5 = (-Alpha - ONE_BY_SQRT3 * Beta) * PWMFullDutyCycle;
		t6 = (Alpha - ONE_BY_SQRT3 * Beta) * PWMFullDutyCycle;

		C = (PWMFullDutyCycle + t5 + t6) / 2;
		A = C - t5;
		B = A - t6;

    case 6
		t6 = (-TWO_BY_SQRT3 * Beta) * PWMFullDutyCycle;
		t1 = (Alpha + ONE_BY_SQRT3 * Beta) * PWMFullDutyCycle;

		A = (PWMFullDutyCycle + t6 + t1) / 2;
		C = A - t1;
		B = C - t6;
end

== matlab function foc_simulink/foc_simulink1/MATLAB Function2 ==
  data: We input; y output; Iq input
function y = fcn(We, Iq)

% y = -We * Lq * Iq;
y = -We * 1.4e-3 * Iq;

== matlab function foc_simulink/foc_simulink1/MATLAB Function3 ==
  data: We input; y output; Id input
function y = fcn(We, Id)

% y = We * (Flux + Ld * Id);  
y = We * (0.034182 + 1.4e-3 * Id);

== matlab function foc_simulink/clarke/MATLAB Function ==
  data: Ia input; Ialpha output; Ib input; Ic input
function Ialpha = fcn(Ia, Ib, Ic)

Ialpha = 3/2 * Ia;

== matlab function foc_simulink/svpwm/svm1 ==
  data: Ualpha input; N output; Ubeta input
function N = fcn(Ualpha, Ubeta)

U1 = Ubeta;
U2 = sqrt(3) * Ualpha - Ubeta;
U3 = -sqrt(3) * Ualpha - Ubeta;
A = 0;
B = 0;
C = 0;

if U1 > 0
    A = 1;
else
    A = 0;
end

if U2 > 0
    B = 1;
else
    B = 0;
end

if U3 > 0
    C = 1;
else
    C = 0;
end

N = A + 2 * B + 4 * C;

== matlab function foc_simulink/svpwm/svm2 ==
  data: Ualpha input; Ubeta input; Tpwm input; Udc input; X output; Y output; Z output
function [X, Y, Z] = fcn(Ualpha, Ubeta, Tpwm, Udc)

X = sqrt(3) * Tpwm * Ubeta / Udc;
Y = sqrt(3) * Tpwm / Udc * (sqrt(3) / 2 * Ualpha + 1 / 2 * Ubeta);
Z = sqrt(3) * Tpwm / Udc * (-sqrt(3) / 2 * Ualpha + 1 / 2 * Ubeta);

== matlab function foc_simulink/svpwm/svm3 ==
  data: N input; T1 output; X input; Y input; Z input; Tpwm input; T2 output
function [T1, T2] = fcn(N, X, Y, Z, Tpwm)

T1 = single(0);
T2 = single(0);

if N == 1
    T1 = Z;
    T2 = Y;
elseif N == 2
    T1 = Y;
    T2 = -X;
elseif N == 3
    T1 = -Z;
    T2 = X;
elseif N == 4
    T1 = -X;
    T2 = Z;
elseif N == 5
    T1 = X;
    T2 = -Y;
elseif N == 6
    T1 = -Y;
    T2 = -Z;
end
